simulink library "linkage_bushing_5DOF_lib"  (R2025a)
settings: Solver=VariableStepAuto  StartTime=0.0  StopTime=10.0  RelTol=1e-3
undefined symbols (not defined in the file): Bushing, Linear, Table, Visual, X, Y, Z
libraries: sm_lib x13, bushing_forces_lib x2
Description:
  | Component of Simscape Vehicle Templates Library
  | 
  | Copyright 2018-2025 The MathWorks, Inc.
settings Model: Creator=smiller  LastModifiedBy=smiller
settings OptimizationCC: ReuseModelBlockBuffer=off
settings ModelReferenceCC: EnableRefExpFcnMdlSchedulingChecks=on
settings RTWCC: GPUComputeCapability=3.5

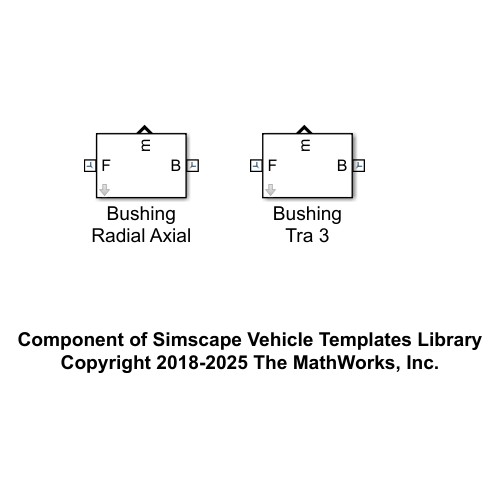
[thumbnail: Simulink's stored preview of the top-level diagram]
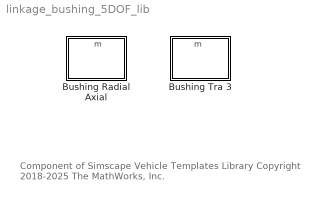
== system linkage_bushing_5DOF_lib ==
  note: Component of Simscape Vehicle Templates Library
      | Copyright 2018-2025 The MathWorks, Inc.
  Bushing Radial Axial : Subsystem  mask(Bushing with Radial and Axial Compliance){checkbox_setTargets=on, popup_force_law_spr_rad=Linear, k_radial=Bushing.RadialSpring.Linear.K.Value, x_radial=Bushing.RadialSpring.Table.x.Value, f_radial_spr=Bushing.RadialSpring.Table.f.Value, k1_radial_max=Bushing.RadialSpring.Maxwell.k1.Value, b1_radial_max=Bushing.RadialSpring.Maxwell.b1.Value, x_radial_max=Bushing.RadialSpring.Maxwell.x.Value, f_radial_max=Bushing.RadialSpring.Maxwell.f.Value, popup_force_law_dam_rad=Linear, d_radial=Bushing.RadialDamper.Linear.d.Value, v_radial=Bushing.RadialDamper.Table.v.Value, f_radial_dam=Bushing.RadialDamper.Table.f.Value, popup_force_law_spr_axi=Table, k_axial=Bushing.AxialSpring.Linear.K.Value, x_axial=Bushing.AxialSpring.Table.x.Value, f_axial_spr=Bushing.AxialSpring.Table.f.Value, popup_force_law_dam_axi=Table, d_axial=Bushing.AxialDamper.Linear.d.Value, v_axial=Bushing.AxialDamper.Linear.v.Value, f_axial_dam=Bushing.AxialDamper.Linear.f.Value, shell_or=Visual.hp.rad*1.05, shell_ir=Visual.hp.rad, shell_len=Visual.hp.rad*4, shell_clr=[0.5 0.5 0.5], shell_opc=1}
      mask prompts: checkbox_setTargets "Set position targets to 0"; popup_force_law_spr_rad "Spring Force Law"; k_radial "Spring Coefficient (N/mm)"; x_radial "Spring Deflection [min max] (mm)"; f_radial_spr "Spring Force [min max] (N)"; k1_radial_max "Maxwell k1"; b1_radial_max "Maxwell b1"; x_radial_max "Maxwell Displacement [min max] (mm)"; f_radial_max "Maxwell Force [min max] (N)"; popup_force_law_dam_rad "Damper Force Law"; d_radial "Damper Coefficient (N/(m/s))"; v_radial "Damper Velocity [min max] (m/s)"; f_radial_dam "Damper Force [min max] (N)"; popup_force_law_spr_axi "Spring Force Law"; k_axial "Spring Coefficient (N/mm)"; x_axial "Spring Displacement [min max] (mm)"; f_axial_spr "Spring Force [min max] (N)"; popup_force_law_dam_axi "Damper Force Law"; d_axial "Damper Coefficient (N/(m/s))"; v_axial "Damper Velocity [min max] (m/s)"; f_axial_dam "Damper Force [min max] (N)"; shell_or "Shell Outer Radius (m)"; shell_ir "Shell Inner Radius (m)"; shell_len "Shell Length (m)"; shell_clr "Shell Color [R G B]"; shell_opc "Shell Opacity [R G B]"
      mask help: Models bushing compliance with independent force laws for radial (x-y plane) and axial (z-axis) directions. Select force laws that model compliance as linear, nonlinear, or nonlinear with hysteresis. Only 5 degrees of freedom are permitted so that the connected part does not rotate about the axis connecting both ends.
      mask init:
      | if(checkbox_setTargets)
      |     set_param([gcb '/Bushing Joint'],...
      |         'PxPositionTargetSpecify','on',...
      |         'PyPositionTargetSpecify','on',...
      |         'PzPositionTargetSpecify','on'...
      |         );
      | else
      |     set_param([gcb '/Bushing Joint'],...
      |         'PxPositionTargetSpecify','off',...
      |         'PyPositionTargetSpecify','off',...
      |         'PzPositionTargetSpecify','off'...
      |         );
      | end
      settings: PortSchema="{\"entries\":[{\"content\":{\"sides\":[{\"content\":{\"connectorIds\":[\"LConn1\"]},\"type\":\"ConnectorPlacement.EquallySpacedRectSide\",\"uuid\":\"540bb151-3239-4a9d-82ba-b7afa97281a8\"},{\"content\":{\"connectorIds\":[\"RConn1\"],\"side\":\"RIGHT\"},\"type\":\"ConnectorPlacement.EquallySpacedRectSide\",\"uuid\":\"0af2999e-e304-4113-9c38-08ac5dd2068d\"},{\"content\":{\"connectorIds\":[\"Out1\"],\"side\":\"TOP\"},\"type\":\"ConnectorPlacement.EquallySpacedRectSide\",\"uuid\":\"c7e19545-6bd3-4656-b994-719fb436eca6\"}]},\"type\":\"ConnectorPlacement.EquallySpacedConnector\",\"uuid\":\"c532a1d4-44be-42d7-8101-c903e69d0a9b\"}],\"packageUris\":[\"http://schema.mathworks.com/mf0/Connector/R2020b\"],\"version\":\"1.0\"}"
      mask TypeOptions popup_force_law_spr_rad: Force Law/popup_force_law_spr_rad
      mask Callback popup_force_law_spr_rad:
      | maskObj = Simulink.Mask.get(gcb); % Get the mask object of the current block
      | krad_h  = maskObj.getParameter('k_radial'); % Get the parameter to hide
      | 
      | xrad_h  = maskObj.getParameter('x_radial'); % Get the parameter to hide
      | fSrad_h = maskObj.getParameter('f_radial_spr'); % Get the parameter to hide
      | k1rad_h  = maskObj.getParameter('k1_radial_max'); % Get the parameter to hide
      | b1rad_h  = maskObj.getParameter('b1_radial_max'); % Get the parameter to hide
      | xmrad_h  = maskObj.getParameter('x_radial_max'); % Get the parameter to hide
      | fmrad_h  = maskObj.getParameter('f_radial_max'); % Get the parameter to hide
      | 
      | % Check the value of ControlParam
      | frcLawSpr = get_param(gcb, 'popup_force_law_spr_rad');
      | 
      | krad_h.Visible  = 'off';
      | xrad_h.Visible  = 'off';
      | fSrad_h.Visible = 'off';
      | k1rad_h.Visible  = 'off';
      | b1rad_h.Visible  = 'off';
      | xmrad_h.Visible  = 'off';
      | fmrad_h.Visible  = 'off';
      | 
      | if strcmp(frcLawSpr, 'Linear')
      |     krad_h.Visible  = 'on';
      | elseif strcmp(frcLawSpr, 'Table')
      |     xrad_h.Visible  = 'on';
      |     fSrad_h.Visible = 'on';
      | elseif strcmp(frcLawSpr, 'Maxwell_SLS')
      |     k1rad_h.Visible  = 'on';
      |     b1rad_h.Visible = 'on';
      |     xmrad_h.Visible = 'on';
      |     fmrad_h.Visible = 'on';
      | end
      mask TypeOptions k_radial: Force Law/k_radial
      mask TypeOptions x_radial: Force Law/x_radial
      mask TypeOptions f_radial_spr: Force Law/f_radial_spr
      mask TypeOptions k1_radial_max: Force Law/k1_radial_max
      mask TypeOptions b1_radial_max: Force Law/b1_radial_max
      mask TypeOptions x_radial_max: Force Law/x_radial_max
      mask TypeOptions f_radial_max: Force Law/f_radial_max
      mask TypeOptions popup_force_law_dam_rad: Force Law/popup_force_law_dam_rad
      mask Callback popup_force_law_dam_rad:
      | maskObj = Simulink.Mask.get(gcb); % Get the mask object of the current block
      | drad_h  = maskObj.getParameter('d_radial'); % Get the parameter to hide
      | 
      | vrad_h  = maskObj.getParameter('v_radial'); % Get the parameter to hide
      | fDrad_h = maskObj.getParameter('f_radial_dam'); % Get the parameter to hide
      | 
      | % Check the value of ControlParam
      | frcLawDam = get_param(gcb, 'popup_force_law_dam_rad');
      | 
      | drad_h.Visible  = 'off';
      | vrad_h.Visible  = 'off';
      | fDrad_h.Visible = 'off';
      | 
      | if strcmp(frcLawDam, 'Linear')
      |     drad_h.Visible  = 'on';
      | elseif strcmp(frcLawDam, 'Table')
      |     vrad_h.Visible  = 'on';
      |     fDrad_h.Visible = 'on';
      | end
      mask TypeOptions d_radial: Force Law/d_radial
      mask TypeOptions v_radial: Force Law/v_radial
      mask TypeOptions f_radial_dam: Force Law/f_radial_dam
      mask TypeOptions popup_force_law_spr_axi: Force Law/popup_force_law_spr_axi
      mask Callback popup_force_law_spr_axi:
      | maskObj = Simulink.Mask.get(gcb); % Get the mask object of the current block
      | kaxi_h  = maskObj.getParameter('k_axial'); % Get the parameter to hide
      | 
      | xaxi_h  = maskObj.getParameter('x_axial'); % Get the parameter to hide
      | fSaxi_h  = maskObj.getParameter('f_axial_spr'); % Get the parameter to hide
      | 
      | % Check the value of ControlParam
      | controlParamValue = get_param(gcb, 'popup_force_law_spr_axi');
      | 
      | kaxi_h.Visible  = 'off';
      | xaxi_h.Visible  = 'off';
      | fSaxi_h.Visible  = 'off';
      | 
      | if strcmp(controlParamValue, 'Linear')
      |     kaxi_h.Visible  = 'on';
      | else
      |     xaxi_h.Visible  = 'on';
      |     fSaxi_h.Visible  = 'on';
      | end
      mask TypeOptions k_axial: Force Law/k_axial
      mask TypeOptions x_axial: Force Law/x_axial
      mask TypeOptions f_axial_spr: Force Law/f_axial_spr
      mask TypeOptions popup_force_law_dam_axi: Force Law/popup_force_law_dam_axi
      mask Callback popup_force_law_dam_axi:
      | maskObj = Simulink.Mask.get(gcb); % Get the mask object of the current block
      | daxi_h  = maskObj.getParameter('d_axial'); % Get the parameter to hide
      | 
      | vaxi_h  = maskObj.getParameter('v_axial'); % Get the parameter to hide
      | fDaxi_h  = maskObj.getParameter('f_axial_dam'); % Get the parameter to hide
      | 
      | % Check the value of ControlParam
      | controlParamValue = get_param(gcb, 'popup_force_law_dam_axi');
      | 
      | daxi_h.Visible  = 'off';
      | vaxi_h.Visible  = 'off';
      | fDaxi_h.Visible  = 'off';
      | 
      | if strcmp(controlParamValue, 'Linear')
      |     daxi_h.Visible  = 'on';
      | else
      |     vaxi_h.Visible  = 'on';
      |     fDaxi_h.Visible  = 'on';
      | end
      mask TypeOptions d_axial: Force Law/d_axial
      mask TypeOptions v_axial: Force Law/v_axial
      mask TypeOptions f_axial_dam: Force Law/f_axial_dam
      mask DialogControl cont_radial Prompt: Radial
      mask DialogControl cont_axial Prompt: Axial
      mask DialogControl cont_vis Prompt: Visualization
  Bushing Tra 3 : Subsystem  mask(Bushing with Independent Axial Compliance on 3 Axes (5 DOF)){checkbox_setTargets=on, popup_force_law_spr_axiX=Linear, k_axialX=Bushing.SpringX.Linear.K.Value, x_axialX=Bushing.SpringX.Table.x.Value, f_axialX_spr=Bushing.SpringX.Table.f.Value, popup_force_law_dam_axiX=Linear, d_axialX=Bushing.DamperX.Linear.d.Value, v_axialX=Bushing.DamperX.Table.v.Value, f_axialX_dam=Bushing.DamperX.Table.f.Value, popup_force_law_spr_axiY=Linear, k_axialY=Bushing.SpringY.Linear.K.Value, x_axialY=Bushing.SpringY.Table.x.Value, f_axialY_spr=Bushing.SpringY.Table.f.Value, popup_force_law_dam_axiY=Linear, d_axialY=Bushing.DamperY.Linear.d.Value, v_axialY=Bushing.DamperY.Table.v.Value, f_axialY_dam=Bushing.DamperY.Table.f.Value, popup_force_law_spr_axiZ=Table, k_axialZ=Bushing.SpringZ.Linear.K.Value, x_axialZ=Bushing.SpringZ.Table.x.Value, f_axialZ_spr=Bushing.SpringZ.Table.f.Value, popup_force_law_dam_axiZ=Table, d_axialZ=Bushing.DamperZ.Linear.d.Value, v_axialZ=Bushing.DamperZ.Table.v.Value, f_axialZ_dam=Bushing.DamperZ.Table.f.Value, shell_or=Visual.hp.rad*2, shell_ir=Visual.hp.rad, shell_len=Visual.hp.rad*2, shell_clr=Visual.Bushing.clr, shell_opc=Visual.part.opc}
      mask prompts: checkbox_setTargets "Set position targets to 0"; popup_force_law_spr_axiX "Spring Force Law"; k_axialX "Spring Coefficient (N/mm)"; x_axialX "Spring Displacement [min max] (mm)"; f_axialX_spr "Spring Force [min max] (N)"; popup_force_law_dam_axiX "Damper Force Law"; d_axialX "Damper Coefficient (N/(m/s))"; v_axialX "Damper Velocity [min max] (m/s)"; f_axialX_dam "Damper Force [min max] (N)"; popup_force_law_spr_axiY "Spring Force Law"; k_axialY "Spring Coefficient (N/mm)"; x_axialY "Spring Displacement [min max] (mm)"; f_axialY_spr "Spring Force [min max] (N)"; popup_force_law_dam_axiY "Damper Force Law"; d_axialY "Damper Coefficient (N/(m/s))"; v_axialY "Damper Velocity [min max] (m/s)"; f_axialY_dam "Damper Force [min max] (N)"; popup_force_law_spr_axiZ "Spring Force Law"; k_axialZ "Spring Coefficient (N/mm)"; x_axialZ "Spring Displacement [min max] (mm)"; f_axialZ_spr "Spring Force [min max] (N)"; popup_force_law_dam_axiZ "Damper Force Law"; d_axialZ "Damper Coefficient (N/(m/s))"; v_axialZ "Damper Velocity [min max] (m/s)"; f_axialZ_dam "Damper Force [min max] (N)"; shell_or "Shell Outer Radius (m)"; shell_ir "Shell Inner Radius (m)"; shell_len "Shell Length (m)"; shell_clr "Shell Color [R G B]"; shell_opc "Shell Opacity [R G B]"
      mask help: Models bushing compliance with independent force laws for x, y, and z directions. Select force laws that model compliance as linear, nonlinear, or nonlinear with hysteresis. Only 5 degrees of freedom are permitted so that the connected part does not rotate about the axis connecting both ends.
      mask init: same as linkage_bushing_5DOF_lib/Bushing Radial Axial
      settings: PortSchema="{\"entries\":[{\"content\":{\"sides\":[{\"content\":{\"connectorIds\":[\"LConn1\"]},\"type\":\"ConnectorPlacement.EquallySpacedRectSide\",\"uuid\":\"540bb151-3239-4a9d-82ba-b7afa97281a8\"},{\"content\":{\"connectorIds\":[\"RConn1\"],\"side\":\"RIGHT\"},\"type\":\"ConnectorPlacement.EquallySpacedRectSide\",\"uuid\":\"0af2999e-e304-4113-9c38-08ac5dd2068d\"},{\"content\":{\"connectorIds\":[\"Out1\"],\"side\":\"TOP\"},\"type\":\"ConnectorPlacement.EquallySpacedRectSide\",\"uuid\":\"c7e19545-6bd3-4656-b994-719fb436eca6\"}]},\"type\":\"ConnectorPlacement.EquallySpacedConnector\",\"uuid\":\"c532a1d4-44be-42d7-8101-c903e69d0a9b\"}],\"packageUris\":[\"http://schema.mathworks.com/mf0/Connector/R2020b\"],\"version\":\"1.0\"}"
      mask TypeOptions popup_force_law_spr_axiX: Force Law/popup_force_law_spr_axiX
      mask Callback popup_force_law_spr_axiX:
      | maskObj = Simulink.Mask.get(gcb); % Get the mask object of the current block
      | kaxiX_h  = maskObj.getParameter('k_axialX'); % Get the parameter to hide
      | 
      | xaxiX_h  = maskObj.getParameter('x_axialX'); % Get the parameter to hide
      | fSaxiX_h  = maskObj.getParameter('f_axialX_spr'); % Get the parameter to hide
      | 
      | % Check the value of ControlParam
      | controlParamValue = get_param(gcb, 'popup_force_law_spr_axiX');
      | 
      | kaxiX_h.Visible  = 'off';
      | xaxiX_h.Visible  = 'off';
      | fSaxiX_h.Visible  = 'off';
      | 
      | if strcmp(controlParamValue, 'Linear')
      |     kaxiX_h.Visible  = 'on';
      | else
      |     xaxiX_h.Visible  = 'on';
      |     fSaxiX_h.Visible  = 'on';
      | end
      mask TypeOptions k_axialX: Force Law/k_axialX
      mask TypeOptions x_axialX: Force Law/x_axialX
      mask TypeOptions f_axialX_spr: Force Law/f_axialX_spr
      mask TypeOptions popup_force_law_dam_axiX: Force Law/popup_force_law_dam_axiX
      mask Callback popup_force_law_dam_axiX:
      | maskObj = Simulink.Mask.get(gcb); % Get the mask object of the current block
      | daxiX_h  = maskObj.getParameter('d_axialX'); % Get the parameter to hide
      | 
      | vaxiX_h  = maskObj.getParameter('v_axialX'); % Get the parameter to hide
      | fDaxiX_h  = maskObj.getParameter('f_axialX_dam'); % Get the parameter to hide
      | 
      | % Check the value of ControlParam
      | controlParamValue = get_param(gcb, 'popup_force_law_dam_axiX');
      | 
      | daxiX_h.Visible  = 'off';
      | vaxiX_h.Visible  = 'off';
      | fDaxiX_h.Visible  = 'off';
      | 
      | if strcmp(controlParamValue, 'Linear')
      |     daxiX_h.Visible  = 'on';
      | else
      |     vaxiX_h.Visible  = 'on';
      |     fDaxiX_h.Visible  = 'on';
      | end
      mask TypeOptions d_axialX: Force Law/d_axialX
      mask TypeOptions v_axialX: Force Law/v_axialX
      mask TypeOptions f_axialX_dam: Force Law/f_axialX_dam
      mask TypeOptions popup_force_law_spr_axiY: Force Law/popup_force_law_spr_axiY
      mask Callback popup_force_law_spr_axiY:
      | maskObj = Simulink.Mask.get(gcb); % Get the mask object of the current block
      | kaxiY_h  = maskObj.getParameter('k_axialY'); % Get the parameter to hide
      | 
      | xaxiY_h  = maskObj.getParameter('x_axialY'); % Get the parameter to hide
      | fSaxiY_h  = maskObj.getParameter('f_axialY_spr'); % Get the parameter to hide
      | 
      | % Check the value of ControlParam
      | controlParamValue = get_param(gcb, 'popup_force_law_spr_axiY');
      | 
      | kaxiY_h.Visible  = 'off';
      | xaxiY_h.Visible  = 'off';
      | fSaxiY_h.Visible  = 'off';
      | 
      | if strcmp(controlParamValue, 'Linear')
      |     kaxiY_h.Visible  = 'on';
      | else
      |     xaxiY_h.Visible  = 'on';
      |     fSaxiY_h.Visible  = 'on';
      | end
      mask TypeOptions k_axialY: Force Law/k_axialY
      mask TypeOptions x_axialY: Force Law/x_axialY
      mask TypeOptions f_axialY_spr: Force Law/f_axialY_spr
      mask TypeOptions popup_force_law_dam_axiY: Force Law/popup_force_law_dam_axiY
      mask Callback popup_force_law_dam_axiY:
      | maskObj = Simulink.Mask.get(gcb); % Get the mask object of the current block
      | daxiY_h  = maskObj.getParameter('d_axialY'); % Get the parameter to hide
      | 
      | vaxiY_h  = maskObj.getParameter('v_axialY'); % Get the parameter to hide
      | fDaxiY_h  = maskObj.getParameter('f_axialY_dam'); % Get the parameter to hide
      | 
      | % Check the value of ControlParam
      | controlParamValue = get_param(gcb, 'popup_force_law_dam_axiY');
      | 
      | daxiY_h.Visible  = 'off';
      | vaxiY_h.Visible  = 'off';
      | fDaxiY_h.Visible  = 'off';
      | 
      | if strcmp(controlParamValue, 'Linear')
      |     daxiY_h.Visible  = 'on';
      | else
      |     vaxiY_h.Visible  = 'on';
      |     fDaxiY_h.Visible  = 'on';
      | end
      mask TypeOptions d_axialY: Force Law/d_axialY
      mask TypeOptions v_axialY: Force Law/v_axialY
      mask TypeOptions f_axialY_dam: Force Law/f_axialY_dam
      mask TypeOptions popup_force_law_spr_axiZ: Force Law/popup_force_law_spr_axiZ
      mask Callback popup_force_law_spr_axiZ:
      | maskObj = Simulink.Mask.get(gcb); % Get the mask object of the current block
      | kaxiZ_h  = maskObj.getParameter('k_axialZ'); % Get the parameter to hide
      | 
      | xaxiZ_h  = maskObj.getParameter('x_axialZ'); % Get the parameter to hide
      | fSaxiZ_h  = maskObj.getParameter('f_axialZ_spr'); % Get the parameter to hide
      | 
      | % Check the value of ControlParam
      | controlParamValue = get_param(gcb, 'popup_force_law_spr_axiZ');
      | 
      | kaxiZ_h.Visible  = 'off';
      | xaxiZ_h.Visible  = 'off';
      | fSaxiZ_h.Visible  = 'off';
      | 
      | if strcmp(controlParamValue, 'Linear')
      |     kaxiZ_h.Visible  = 'on';
      | else
      |     xaxiZ_h.Visible  = 'on';
      |     fSaxiZ_h.Visible  = 'on';
      | end
      mask TypeOptions k_axialZ: Force Law/k_axialZ
      mask TypeOptions x_axialZ: Force Law/x_axialZ
      mask TypeOptions f_axialZ_spr: Force Law/f_axialZ_spr
      mask TypeOptions popup_force_law_dam_axiZ: Force Law/popup_force_law_dam_axiZ
      mask Callback popup_force_law_dam_axiZ:
      | maskObj = Simulink.Mask.get(gcb); % Get the mask object of the current block
      | daxiZ_h  = maskObj.getParameter('d_axialZ'); % Get the parameter to hide
      | 
      | vaxiZ_h  = maskObj.getParameter('v_axialZ'); % Get the parameter to hide
      | fDaxiZ_h  = maskObj.getParameter('f_axialZ_dam'); % Get the parameter to hide
      | 
      | % Check the value of ControlParam
      | controlParamValue = get_param(gcb, 'popup_force_law_dam_axiZ');
      | 
      | daxiZ_h.Visible  = 'off';
      | vaxiZ_h.Visible  = 'off';
      | fDaxiZ_h.Visible  = 'off';
      | 
      | if strcmp(controlParamValue, 'Linear')
      |     daxiZ_h.Visible  = 'on';
      | else
      |     vaxiZ_h.Visible  = 'on';
      |     fDaxiZ_h.Visible  = 'on';
      | end
      mask TypeOptions d_axialZ: Force Law/d_axialZ
      mask TypeOptions v_axialZ: Force Law/v_axialZ
      mask TypeOptions f_axialZ_dam: Force Law/f_axialZ_dam
      mask DialogControl cont_axialX Prompt: Axial (local x)
      mask DialogControl cont_axialY Prompt: Axial (local y)
      mask DialogControl cont_axialZ Prompt: Axial (local z)
      mask DialogControl cont_vis Prompt: Visualization

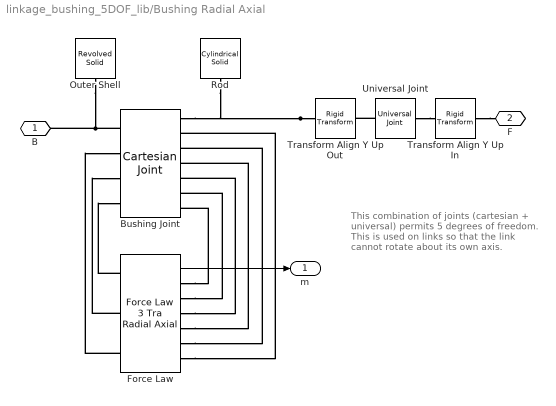
== system linkage_bushing_5DOF_lib/Bushing Radial Axial ==
  note: This combination of joints (cartesian + universal) permits 5 degrees of freedom. This is used on links so that the link cannot rotate about its own axis.
  Bushing Joint : sm_lib/Joints/Cartesian Joint  JointMode=Normal  CompositeWrenchDir=FollowerOnBase  CompositeWrenchFrame=BaseFrame  SenseConstraintForce=off  SenseConstraintTorque=off  SenseTotalForce=off  SenseTotalTorque=off  PxPositionTargetSpecify=on  PxPositionTargetPriority=High  PxPositionTargetValue=0  PxPositionTargetValueUnits=m  PxVelocityTargetSpecify=off  PxVelocityTargetPriority=High  PxVelocityTargetValue=0  PxVelocityTargetValueUnits=m/s  PxEquilibriumPosition=0  PxEquilibriumPositionUnits=m  PxSpringStiffness=0  PxSpringStiffnessUnits=N/m  PxDampingCoefficient=0  PxDampingCoefficientUnits=N/(m/s)  PxLowerLimitSpecify=off  PxLowerLimitBound=-1  PxLowerLimitBoundUnits=m  PxLowerLimitStiffness=1e6  PxLowerLimitStiffnessUnits=N/m  PxLowerLimitDamping=1e3  PxLowerLimitDampingUnits=N/(m/s)  PxLowerLimitTransitionRegionWidth=1e-4  PxLowerLimitTransitionRegionWidthUnits=m  PxUpperLimitSpecify=off  PxUpperLimitBound=1  PxUpperLimitBoundUnits=m  PxUpperLimitStiffness=1e6  PxUpperLimitStiffnessUnits=N/m  PxUpperLimitDamping=1e3  PxUpperLimitDampingUnits=N/(m/s)  PxUpperLimitTransitionRegionWidth=1e-4  PxUpperLimitTransitionRegionWidthUnits=m  PxTorqueActuationMode=InputTorque  PxMotionActuationMode=ComputedMotion  PxSensePosition=on  PxSenseVelocity=on  PxSenseAcceleration=off  PxSenseTorqueForce=off  PxSenseLowerLimitTorqueForce=off  PxSenseUpperLimitTorqueForce=off  PyPositionTargetSpecify=on  PyPositionTargetPriority=High  PyPositionTargetValue=0  PyPositionTargetValueUnits=m  PyVelocityTargetSpecify=off  PyVelocityTargetPriority=High  PyVelocityTargetValue=0  PyVelocityTargetValueUnits=m/s  PyEquilibriumPosition=0  PyEquilibriumPositionUnits=m  PySpringStiffness=0  PySpringStiffnessUnits=N/m  PyDampingCoefficient=0  PyDampingCoefficientUnits=N/(m/s)  PyLowerLimitSpecify=off  PyLowerLimitBound=-1  PyLowerLimitBoundUnits=m  PyLowerLimitStiffness=1e6  PyLowerLimitStiffnessUnits=N/m  PyLowerLimitDamping=1e3  PyLowerLimitDampingUnits=N/(m/s)  PyLowerLimitTransitionRegionWidth=1e-4  PyLowerLimitTransitionRegionWidthUnits=m  PyUpperLimitSpecify=off  PyUpperLimitBound=1  PyUpperLimitBoundUnits=m  PyUpperLimitStiffness=1e6  PyUpperLimitStiffnessUnits=N/m  PyUpperLimitDamping=1e3  PyUpperLimitDampingUnits=N/(m/s)  PyUpperLimitTransitionRegionWidth=1e-4  PyUpperLimitTransitionRegionWidthUnits=m  PyTorqueActuationMode=InputTorque  PyMotionActuationMode=ComputedMotion  PySensePosition=on  PySenseVelocity=on  PySenseAcceleration=off  PySenseTorqueForce=off  PySenseLowerLimitTorqueForce=off  PySenseUpperLimitTorqueForce=off  PzPositionTargetSpecify=on  PzPositionTargetPriority=High  PzPositionTargetValue=0  PzPositionTargetValueUnits=m  PzVelocityTargetSpecify=off  PzVelocityTargetPriority=High  PzVelocityTargetValue=0  PzVelocityTargetValueUnits=m/s  PzEquilibriumPosition=0  PzEquilibriumPositionUnits=m  PzSpringStiffness=0  PzSpringStiffnessUnits=N/m  PzDampingCoefficient=0  PzDampingCoefficientUnits=N/(m/s)  PzLowerLimitSpecify=off  PzLowerLimitBound=-1  PzLowerLimitBoundUnits=m  PzLowerLimitStiffness=1e6  PzLowerLimitStiffnessUnits=N/m  PzLowerLimitDamping=1e3  PzLowerLimitDampingUnits=N/(m/s)  PzLowerLimitTransitionRegionWidth=1e-4  PzLowerLimitTransitionRegionWidthUnits=m  PzUpperLimitSpecify=off  PzUpperLimitBound=1  PzUpperLimitBoundUnits=m  PzUpperLimitStiffness=1e6  PzUpperLimitStiffnessUnits=N/m  PzUpperLimitDamping=1e3  PzUpperLimitDampingUnits=N/(m/s)  PzUpperLimitTransitionRegionWidth=1e-4  PzUpperLimitTransitionRegionWidthUnits=m  PzTorqueActuationMode=InputTorque  PzMotionActuationMode=ComputedMotion  PzSensePosition=on  PzSenseVelocity=on  PzSenseAcceleration=off  PzSenseTorqueForce=off  PzSenseLowerLimitTorqueForce=off  PzSenseUpperLimitTorqueForce=off
  Force Law : bushing_forces_lib/Force Law 3 Tra Radial Axial  popup_force_law_spr_rad=Linear  k_radial=k_radial  x_radial=x_radial  f_radial_spr=f_radial_spr  k1_radial_max=k1_radial_max  b1_radial_max=b1_radial_max  x_radial_max=x_radial_max  f_radial_max=f_radial_max  popup_force_law_dam_rad=Linear  d_radial=d_radial  v_radial=v_radial  f_radial_dam=f_radial_dam  popup_force_law_spr_axi=Table  k_axial=k_axial  x_axial=x_axial  f_axial_spr=f_axial_spr  popup_force_law_dam_axi=Table  d_axial=d_axial  v_axial=v_axial  f_axial_dam=f_axial_dam
  Outer Shell : sm_lib/Body Elements/Revolved Solid  RevolutionCrossSection=[shell_ir 0.5; shell_ir -0.5; shell_or -0.5; shell_or 0.5].*[1 shell_len]  RevolutionCrossSectionUnits=m  RevolutionExtent=Full  RevolutionAngle=180  RevolutionAngleUnits=deg  ExportConvexHullGeometry=off  InertiaType=CalculateFromGeometry  BasedOnType=Density  Density=1  DensityUnits=kg/m^3  Mass=1  MassUnits=kg  CenterOfMass=[0 0 0]  CenterOfMassUnits=m  MomentsOfInertia=[1 1 1]  MomentsOfInertiaUnits=kg*m^2  ProductsOfInertia=[0 0 0]  ProductsOfInertiaUnits=kg*m^2  GraphicType=FromGeometry  MarkerShape=Sphere  MarkerSize=10  GraphicVisPropType=SimpleVisualProperties  GraphicDiffuseColor=shell_clr  GraphicOpacity=shell_opc  GraphicSpecularColor=[0.5 0.5 0.5 1.0]  GraphicAmbientColor=[0.15 0.15 0.15 1.0]  GraphicEmissiveColor=[0.0 0.0 0.0 1.0]  GraphicShininess=75  DoExposeReferenceFrame=on  SerializedFrames=<Frames/>
  Rod : sm_lib/Body Elements/Cylindrical Solid  CylinderRadius=shell_ir/2  CylinderRadiusUnits=m  CylinderLength=shell_len  CylinderLengthUnits=m  ExportEntireGeometry=off  InertiaType=CalculateFromGeometry  BasedOnType=Density  Density=1  DensityUnits=kg/m^3  Mass=1  MassUnits=kg  CenterOfMass=[0 0 0]  CenterOfMassUnits=m  MomentsOfInertia=[1 1 1]  MomentsOfInertiaUnits=kg*m^2  ProductsOfInertia=[0 0 0]  ProductsOfInertiaUnits=kg*m^2  GraphicType=FromGeometry  MarkerShape=Sphere  MarkerSize=10  GraphicVisPropType=SimpleVisualProperties  GraphicDiffuseColor=shell_clr  GraphicOpacity=shell_opc  GraphicSpecularColor=[0.5 0.5 0.5 1.0]  GraphicAmbientColor=[0.15 0.15 0.15 1.0]  GraphicEmissiveColor=[0.0 0.0 0.0 1.0]  GraphicShininess=75  DoExposeReferenceFrame=on  SerializedFrames=<Frames/>
  Transform Align Y Up In : sm_lib/Frames and Transforms/Rigid Transform  RotationMethod=StandardAxis  FollAlignAxisA=+X  BaseAlignAxisA=+Y  FollAlignAxisB=+Y  BaseAlignAxisB=+Z  RotationStandardAxis=+X  RotationAngle=90  RotationAngleUnits=deg  RotationArbitraryAxis=[0 0 1]  RotationSequenceAxes=FollowerAxes  RotationSequence=XYX  RotationSequenceAngles=[0 0 0]  RotationSequenceAnglesUnits=deg  RotationMatrix=[1 0 0; 0 1 0; 0 0 1]  Quaternion=[1 0 0 0]  TranslationMethod=None  TranslationCartesianOffset=[0 0 0]  TranslationCartesianOffsetUnits=m  TranslationStandardAxis=+Z  TranslationStandardOffset=0  TranslationStandardOffsetUnits=m  TranslationROffset=0  TranslationROffsetUnits=m  TranslationThetaOffset=0  TranslationThetaOffsetUnits=deg  TranslationZOffset=0  TranslationZOffsetUnits=m
  Transform Align Y Up Out : sm_lib/Frames and Transforms/Rigid Transform  RotationMethod=StandardAxis  FollAlignAxisA=+X  BaseAlignAxisA=+Y  FollAlignAxisB=+Y  BaseAlignAxisB=+Z  RotationStandardAxis=+X  RotationAngle=90  RotationAngleUnits=deg  RotationArbitraryAxis=[0 0 1]  RotationSequenceAxes=FollowerAxes  RotationSequence=XYX  RotationSequenceAngles=[0 0 0]  RotationSequenceAnglesUnits=deg  RotationMatrix=[1 0 0; 0 1 0; 0 0 1]  Quaternion=[1 0 0 0]  TranslationMethod=None  TranslationCartesianOffset=[0 0 0]  TranslationCartesianOffsetUnits=m  TranslationStandardAxis=+Z  TranslationStandardOffset=0  TranslationStandardOffsetUnits=m  TranslationROffset=0  TranslationROffsetUnits=m  TranslationThetaOffset=0  TranslationThetaOffsetUnits=deg  TranslationZOffset=0  TranslationZOffsetUnits=m
  Universal Joint : sm_lib/Joints/Universal Joint  JointMode=Normal  CompositeWrenchDir=FollowerOnBase  CompositeWrenchFrame=BaseFrame  SenseConstraintForce=off  SenseConstraintTorque=off  SenseTotalForce=off  SenseTotalTorque=off  RxPositionTargetSpecify=off  RxPositionTargetPriority=High  RxPositionTargetValue=0  RxPositionTargetValueUnits=deg  RxVelocityTargetSpecify=off  RxVelocityTargetPriority=High  RxVelocityTargetValue=0  RxVelocityTargetValueUnits=deg/s  RxEquilibriumPosition=0  RxEquilibriumPositionUnits=deg  RxSpringStiffness=0  RxSpringStiffnessUnits=N*m/deg  RxDampingCoefficient=0  RxDampingCoefficientUnits=N*m/(deg/s)  RxLowerLimitSpecify=off  RxLowerLimitBound=-90  RxLowerLimitBoundUnits=deg  RxLowerLimitStiffness=1e4  RxLowerLimitStiffnessUnits=N*m/deg  RxLowerLimitDamping=10  RxLowerLimitDampingUnits=N*m/(deg/s)  RxLowerLimitTransitionRegionWidth=0.1  RxLowerLimitTransitionRegionWidthUnits=deg  RxUpperLimitSpecify=off  RxUpperLimitBound=90  RxUpperLimitBoundUnits=deg  RxUpperLimitStiffness=1e4  RxUpperLimitStiffnessUnits=N*m/deg  RxUpperLimitDamping=10  RxUpperLimitDampingUnits=N*m/(deg/s)  RxUpperLimitTransitionRegionWidth=0.1  RxUpperLimitTransitionRegionWidthUnits=deg  RxTorqueActuationMode=NoTorque  RxMotionActuationMode=ComputedMotion  RxSensePosition=off  RxSenseVelocity=off  RxSenseAcceleration=off  RxSenseTorqueForce=off  RxSenseLowerLimitTorqueForce=off  RxSenseUpperLimitTorqueForce=off  RyPositionTargetSpecify=off  RyPositionTargetPriority=High  RyPositionTargetValue=0  RyPositionTargetValueUnits=deg  RyVelocityTargetSpecify=off  RyVelocityTargetPriority=High  RyVelocityTargetValue=0  RyVelocityTargetValueUnits=deg/s  RyEquilibriumPosition=0  RyEquilibriumPositionUnits=deg  RySpringStiffness=0  RySpringStiffnessUnits=N*m/deg  RyDampingCoefficient=0  RyDampingCoefficientUnits=N*m/(deg/s)  RyLowerLimitSpecify=off  RyLowerLimitBound=-90  RyLowerLimitBoundUnits=deg  RyLowerLimitStiffness=1e4  RyLowerLimitStiffnessUnits=N*m/deg  RyLowerLimitDamping=10  RyLowerLimitDampingUnits=N*m/(deg/s)  RyLowerLimitTransitionRegionWidth=0.1  RyLowerLimitTransitionRegionWidthUnits=deg  RyUpperLimitSpecify=off  RyUpperLimitBound=90  RyUpperLimitBoundUnits=deg  RyUpperLimitStiffness=1e4  RyUpperLimitStiffnessUnits=N*m/deg  RyUpperLimitDamping=10  RyUpperLimitDampingUnits=N*m/(deg/s)  RyUpperLimitTransitionRegionWidth=0.1  RyUpperLimitTransitionRegionWidthUnits=deg  RyTorqueActuationMode=NoTorque  RyMotionActuationMode=ComputedMotion  RySensePosition=off  RySenseVelocity=off  RySenseAcceleration=off  RySenseTorqueForce=off  RySenseLowerLimitTorqueForce=off  RySenseUpperLimitTorqueForce=off
  B : PMIOPort  Side=Left
  F : PMIOPort  Port=2  Side=Right
  m : Outport
  wires:
  Force Law/1 -> m/1
  connections:
  Force Law/LConn2 -- Bushing Joint/LConn3
  Force Law/RConn5 -- Bushing Joint/RConn3
  Force Law/LConn3 -- Bushing Joint/LConn2
  Force Law/LConn1 -- Bushing Joint/LConn4
  Force Law/RConn1 -- Bushing Joint/RConn7
  Force Law/RConn3 -- Bushing Joint/RConn5
  Force Law/RConn2 -- Bushing Joint/RConn6
  Force Law/RConn4 -- Bushing Joint/RConn4
  Force Law/RConn6 -- Bushing Joint/RConn2
  Transform Align Y Up Out/LConn1 -- Bushing Joint/RConn1 -- Rod/RConn1
  Universal Joint/LConn1 -- Transform Align Y Up Out/RConn1
  Universal Joint/RConn1 -- Transform Align Y Up In/RConn1
  Outer Shell/RConn1 -- B/RConn1 -- Bushing Joint/LConn1
  Transform Align Y Up In/LConn1 -- F/RConn1

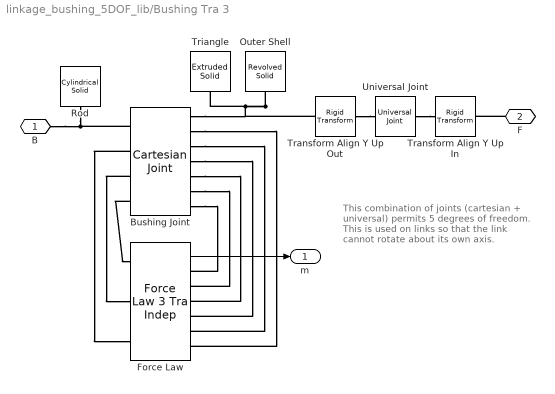
== system linkage_bushing_5DOF_lib/Bushing Tra 3 ==
  note: This combination of joints (cartesian + universal) permits 5 degrees of freedom. This is used on links so that the link cannot rotate about its own axis.
  Bushing Joint : sm_lib/Joints/Cartesian Joint  JointMode=Normal  CompositeWrenchDir=FollowerOnBase  CompositeWrenchFrame=BaseFrame  SenseConstraintForce=off  SenseConstraintTorque=off  SenseTotalForce=off  SenseTotalTorque=off  PxPositionTargetSpecify=on  PxPositionTargetPriority=High  PxPositionTargetValue=0  PxPositionTargetValueUnits=m  PxVelocityTargetSpecify=off  PxVelocityTargetPriority=High  PxVelocityTargetValue=0  PxVelocityTargetValueUnits=m/s  PxEquilibriumPosition=0  PxEquilibriumPositionUnits=m  PxSpringStiffness=0  PxSpringStiffnessUnits=N/m  PxDampingCoefficient=0  PxDampingCoefficientUnits=N/(m/s)  PxLowerLimitSpecify=off  PxLowerLimitBound=-1  PxLowerLimitBoundUnits=m  PxLowerLimitStiffness=1e6  PxLowerLimitStiffnessUnits=N/m  PxLowerLimitDamping=1e3  PxLowerLimitDampingUnits=N/(m/s)  PxLowerLimitTransitionRegionWidth=1e-4  PxLowerLimitTransitionRegionWidthUnits=m  PxUpperLimitSpecify=off  PxUpperLimitBound=1  PxUpperLimitBoundUnits=m  PxUpperLimitStiffness=1e6  PxUpperLimitStiffnessUnits=N/m  PxUpperLimitDamping=1e3  PxUpperLimitDampingUnits=N/(m/s)  PxUpperLimitTransitionRegionWidth=1e-4  PxUpperLimitTransitionRegionWidthUnits=m  PxTorqueActuationMode=InputTorque  PxMotionActuationMode=ComputedMotion  PxSensePosition=on  PxSenseVelocity=on  PxSenseAcceleration=off  PxSenseTorqueForce=off  PxSenseLowerLimitTorqueForce=off  PxSenseUpperLimitTorqueForce=off  PyPositionTargetSpecify=on  PyPositionTargetPriority=High  PyPositionTargetValue=0  PyPositionTargetValueUnits=m  PyVelocityTargetSpecify=off  PyVelocityTargetPriority=High  PyVelocityTargetValue=0  PyVelocityTargetValueUnits=m/s  PyEquilibriumPosition=0  PyEquilibriumPositionUnits=m  PySpringStiffness=0  PySpringStiffnessUnits=N/m  PyDampingCoefficient=0  PyDampingCoefficientUnits=N/(m/s)  PyLowerLimitSpecify=off  PyLowerLimitBound=-1  PyLowerLimitBoundUnits=m  PyLowerLimitStiffness=1e6  PyLowerLimitStiffnessUnits=N/m  PyLowerLimitDamping=1e3  PyLowerLimitDampingUnits=N/(m/s)  PyLowerLimitTransitionRegionWidth=1e-4  PyLowerLimitTransitionRegionWidthUnits=m  PyUpperLimitSpecify=off  PyUpperLimitBound=1  PyUpperLimitBoundUnits=m  PyUpperLimitStiffness=1e6  PyUpperLimitStiffnessUnits=N/m  PyUpperLimitDamping=1e3  PyUpperLimitDampingUnits=N/(m/s)  PyUpperLimitTransitionRegionWidth=1e-4  PyUpperLimitTransitionRegionWidthUnits=m  PyTorqueActuationMode=InputTorque  PyMotionActuationMode=ComputedMotion  PySensePosition=on  PySenseVelocity=on  PySenseAcceleration=off  PySenseTorqueForce=off  PySenseLowerLimitTorqueForce=off  PySenseUpperLimitTorqueForce=off  PzPositionTargetSpecify=on  PzPositionTargetPriority=High  PzPositionTargetValue=0  PzPositionTargetValueUnits=m  PzVelocityTargetSpecify=off  PzVelocityTargetPriority=High  PzVelocityTargetValue=0  PzVelocityTargetValueUnits=m/s  PzEquilibriumPosition=0  PzEquilibriumPositionUnits=m  PzSpringStiffness=0  PzSpringStiffnessUnits=N/m  PzDampingCoefficient=0  PzDampingCoefficientUnits=N/(m/s)  PzLowerLimitSpecify=off  PzLowerLimitBound=-1  PzLowerLimitBoundUnits=m  PzLowerLimitStiffness=1e6  PzLowerLimitStiffnessUnits=N/m  PzLowerLimitDamping=1e3  PzLowerLimitDampingUnits=N/(m/s)  PzLowerLimitTransitionRegionWidth=1e-4  PzLowerLimitTransitionRegionWidthUnits=m  PzUpperLimitSpecify=off  PzUpperLimitBound=1  PzUpperLimitBoundUnits=m  PzUpperLimitStiffness=1e6  PzUpperLimitStiffnessUnits=N/m  PzUpperLimitDamping=1e3  PzUpperLimitDampingUnits=N/(m/s)  PzUpperLimitTransitionRegionWidth=1e-4  PzUpperLimitTransitionRegionWidthUnits=m  PzTorqueActuationMode=InputTorque  PzMotionActuationMode=ComputedMotion  PzSensePosition=on  PzSenseVelocity=on  PzSenseAcceleration=off  PzSenseTorqueForce=off  PzSenseLowerLimitTorqueForce=off  PzSenseUpperLimitTorqueForce=off
  Force Law : bushing_forces_lib/Force Law 3 Tra Indep  popup_force_law_spr_axiX=Linear  k_axialX=k_axialX  x_axialX=x_axialX  f_axialX_spr=f_axialX_spr  popup_force_law_dam_axiX=Linear  d_axialX=d_axialX  v_axialX=v_axialX  f_axialX_dam=f_axialX_dam  popup_force_law_spr_axiY=Linear  k_axialY=k_axialY  x_axialY=x_axialY  f_axialY_spr=f_axialY_spr  popup_force_law_dam_axiY=Linear  d_axialY=d_axialY  v_axialY=v_axialY  f_axialY_dam=f_axialY_dam  popup_force_law_spr_axiZ=Table  k_axialZ=k_axialZ  x_axialZ=x_axialZ  f_axialZ_spr=f_axialZ_spr  popup_force_law_dam_axiZ=Table  d_axialZ=d_axialZ  f_axialZ_dam=f_axialZ_dam  v_axialZ=v_axialZ
  Outer Shell : sm_lib/Body Elements/Revolved Solid  RevolutionCrossSection=[shell_ir 0.5; shell_ir -0.5; shell_or -0.5; shell_or 0.5].*[1 shell_len]  RevolutionCrossSectionUnits=m  RevolutionExtent=Full  RevolutionAngle=180  RevolutionAngleUnits=deg  ExportConvexHullGeometry=off  InertiaType=CalculateFromGeometry  BasedOnType=Density  Density=1  DensityUnits=kg/m^3  Mass=1  MassUnits=kg  CenterOfMass=[0 0 0]  CenterOfMassUnits=m  MomentsOfInertia=[1 1 1]  MomentsOfInertiaUnits=kg*m^2  ProductsOfInertia=[0 0 0]  ProductsOfInertiaUnits=kg*m^2  GraphicType=FromGeometry  MarkerShape=Sphere  MarkerSize=10  GraphicVisPropType=SimpleVisualProperties  GraphicDiffuseColor=shell_clr  GraphicOpacity=shell_opc  GraphicSpecularColor=[0.5 0.5 0.5 1.0]  GraphicAmbientColor=[0.15 0.15 0.15 1.0]  GraphicEmissiveColor=[0.0 0.0 0.0 1.0]  GraphicShininess=75  DoExposeReferenceFrame=on  SerializedFrames=<Frames/>
  Rod : sm_lib/Body Elements/Cylindrical Solid  CylinderRadius=shell_ir/2  CylinderRadiusUnits=m  CylinderLength=shell_len  CylinderLengthUnits=m  ExportEntireGeometry=off  InertiaType=CalculateFromGeometry  BasedOnType=Density  Density=1  DensityUnits=kg/m^3  Mass=1  MassUnits=kg  CenterOfMass=[0 0 0]  CenterOfMassUnits=m  MomentsOfInertia=[1 1 1]  MomentsOfInertiaUnits=kg*m^2  ProductsOfInertia=[0 0 0]  ProductsOfInertiaUnits=kg*m^2  GraphicType=FromGeometry  MarkerShape=Sphere  MarkerSize=10  GraphicVisPropType=SimpleVisualProperties  GraphicDiffuseColor=shell_clr  GraphicOpacity=shell_opc  GraphicSpecularColor=[0.5 0.5 0.5 1.0]  GraphicAmbientColor=[0.15 0.15 0.15 1.0]  GraphicEmissiveColor=[0.0 0.0 0.0 1.0]  GraphicShininess=75  DoExposeReferenceFrame=on  SerializedFrames=<Frames/>
  Transform Align Y Up In : sm_lib/Frames and Transforms/Rigid Transform  RotationMethod=StandardAxis  FollAlignAxisA=+X  BaseAlignAxisA=+Y  FollAlignAxisB=+Y  BaseAlignAxisB=+Z  RotationStandardAxis=+X  RotationAngle=90  RotationAngleUnits=deg  RotationArbitraryAxis=[0 0 1]  RotationSequenceAxes=FollowerAxes  RotationSequence=XYX  RotationSequenceAngles=[0 0 0]  RotationSequenceAnglesUnits=deg  RotationMatrix=[1 0 0; 0 1 0; 0 0 1]  Quaternion=[1 0 0 0]  TranslationMethod=None  TranslationCartesianOffset=[0 0 0]  TranslationCartesianOffsetUnits=m  TranslationStandardAxis=+Z  TranslationStandardOffset=0  TranslationStandardOffsetUnits=m  TranslationROffset=0  TranslationROffsetUnits=m  TranslationThetaOffset=0  TranslationThetaOffsetUnits=deg  TranslationZOffset=0  TranslationZOffsetUnits=m
  Transform Align Y Up Out : sm_lib/Frames and Transforms/Rigid Transform  RotationMethod=StandardAxis  FollAlignAxisA=+X  BaseAlignAxisA=+Y  FollAlignAxisB=+Y  BaseAlignAxisB=+Z  RotationStandardAxis=+X  RotationAngle=90  RotationAngleUnits=deg  RotationArbitraryAxis=[0 0 1]  RotationSequenceAxes=FollowerAxes  RotationSequence=XYX  RotationSequenceAngles=[0 0 0]  RotationSequenceAnglesUnits=deg  RotationMatrix=[1 0 0; 0 1 0; 0 0 1]  Quaternion=[1 0 0 0]  TranslationMethod=None  TranslationCartesianOffset=[0 0 0]  TranslationCartesianOffsetUnits=m  TranslationStandardAxis=+Z  TranslationStandardOffset=0  TranslationStandardOffsetUnits=m  TranslationROffset=0  TranslationROffsetUnits=m  TranslationThetaOffset=0  TranslationThetaOffsetUnits=deg  TranslationZOffset=0  TranslationZOffsetUnits=m
  Triangle : sm_lib/Body Elements/Extruded Solid  ExtrusionType=General  PolygonNumSides=3  PolygonOuterRadius=1  PolygonOuterRadiusUnits=m  ExportEntireGeometry=off  ExtrusionCrossSection=[cosd(-70) sind(-70);1 0;cosd(70) sind(70)]*shell_or  ExtrusionCrossSectionUnits=m  ExportConvexHullGeometry=off  ExtrusionLength=shell_len+0.001  ExtrusionLengthUnits=m  InertiaType=CalculateFromGeometry  BasedOnType=Density  Density=1  DensityUnits=kg/m^3  Mass=1  MassUnits=kg  CenterOfMass=[0 0 0]  CenterOfMassUnits=m  MomentsOfInertia=[1 1 1]  MomentsOfInertiaUnits=kg*m^2  ProductsOfInertia=[0 0 0]  ProductsOfInertiaUnits=kg*m^2  GraphicType=FromGeometry  MarkerShape=Sphere  MarkerSize=10  GraphicVisPropType=SimpleVisualProperties  GraphicDiffuseColor=[0.6 1.0 0.0]  GraphicOpacity=1.0  GraphicSpecularColor=[0.5 0.5 0.5 1.0]  GraphicAmbientColor=[0.15 0.15 0.15 1.0]  GraphicEmissiveColor=[0.0 0.0 0.0 1.0]  GraphicShininess=75  DoExposeReferenceFrame=on  SerializedFrames=<Frames/>
  Universal Joint : sm_lib/Joints/Universal Joint  JointMode=Normal  CompositeWrenchDir=FollowerOnBase  CompositeWrenchFrame=BaseFrame  SenseConstraintForce=off  SenseConstraintTorque=off  SenseTotalForce=off  SenseTotalTorque=off  RxPositionTargetSpecify=off  RxPositionTargetPriority=High  RxPositionTargetValue=0  RxPositionTargetValueUnits=deg  RxVelocityTargetSpecify=off  RxVelocityTargetPriority=High  RxVelocityTargetValue=0  RxVelocityTargetValueUnits=deg/s  RxEquilibriumPosition=0  RxEquilibriumPositionUnits=deg  RxSpringStiffness=0  RxSpringStiffnessUnits=N*m/deg  RxDampingCoefficient=0  RxDampingCoefficientUnits=N*m/(deg/s)  RxLowerLimitSpecify=off  RxLowerLimitBound=-90  RxLowerLimitBoundUnits=deg  RxLowerLimitStiffness=1e4  RxLowerLimitStiffnessUnits=N*m/deg  RxLowerLimitDamping=10  RxLowerLimitDampingUnits=N*m/(deg/s)  RxLowerLimitTransitionRegionWidth=0.1  RxLowerLimitTransitionRegionWidthUnits=deg  RxUpperLimitSpecify=off  RxUpperLimitBound=90  RxUpperLimitBoundUnits=deg  RxUpperLimitStiffness=1e4  RxUpperLimitStiffnessUnits=N*m/deg  RxUpperLimitDamping=10  RxUpperLimitDampingUnits=N*m/(deg/s)  RxUpperLimitTransitionRegionWidth=0.1  RxUpperLimitTransitionRegionWidthUnits=deg  RxTorqueActuationMode=NoTorque  RxMotionActuationMode=ComputedMotion  RxSensePosition=off  RxSenseVelocity=off  RxSenseAcceleration=off  RxSenseTorqueForce=off  RxSenseLowerLimitTorqueForce=off  RxSenseUpperLimitTorqueForce=off  RyPositionTargetSpecify=off  RyPositionTargetPriority=High  RyPositionTargetValue=0  RyPositionTargetValueUnits=deg  RyVelocityTargetSpecify=off  RyVelocityTargetPriority=High  RyVelocityTargetValue=0  RyVelocityTargetValueUnits=deg/s  RyEquilibriumPosition=0  RyEquilibriumPositionUnits=deg  RySpringStiffness=0  RySpringStiffnessUnits=N*m/deg  RyDampingCoefficient=0  RyDampingCoefficientUnits=N*m/(deg/s)  RyLowerLimitSpecify=off  RyLowerLimitBound=-90  RyLowerLimitBoundUnits=deg  RyLowerLimitStiffness=1e4  RyLowerLimitStiffnessUnits=N*m/deg  RyLowerLimitDamping=10  RyLowerLimitDampingUnits=N*m/(deg/s)  RyLowerLimitTransitionRegionWidth=0.1  RyLowerLimitTransitionRegionWidthUnits=deg  RyUpperLimitSpecify=off  RyUpperLimitBound=90  RyUpperLimitBoundUnits=deg  RyUpperLimitStiffness=1e4  RyUpperLimitStiffnessUnits=N*m/deg  RyUpperLimitDamping=10  RyUpperLimitDampingUnits=N*m/(deg/s)  RyUpperLimitTransitionRegionWidth=0.1  RyUpperLimitTransitionRegionWidthUnits=deg  RyTorqueActuationMode=NoTorque  RyMotionActuationMode=ComputedMotion  RySensePosition=off  RySenseVelocity=off  RySenseAcceleration=off  RySenseTorqueForce=off  RySenseLowerLimitTorqueForce=off  RySenseUpperLimitTorqueForce=off
  B : PMIOPort  Side=Left
  F : PMIOPort  Port=2  Side=Right
  m : Outport
  wires:
  Force Law/1 -> m/1
  connections:
  Bushing Joint/LConn3 -- Force Law/LConn2
  Outer Shell/RConn1 -- Bushing Joint/RConn1 -- Transform Align Y Up Out/LConn1 -- Triangle/RConn1
  Bushing Joint/RConn3 -- Force Law/RConn5
  Bushing Joint/LConn2 -- Force Law/LConn3
  Bushing Joint/LConn4 -- Force Law/LConn1
  Bushing Joint/RConn7 -- Force Law/RConn1
  Bushing Joint/RConn5 -- Force Law/RConn3
  Bushing Joint/RConn6 -- Force Law/RConn2
  Bushing Joint/RConn4 -- Force Law/RConn4
  Bushing Joint/RConn2 -- Force Law/RConn6
  Rod/RConn1 -- Bushing Joint/LConn1 -- B/RConn1
  Transform Align Y Up Out/RConn1 -- Universal Joint/LConn1
  Universal Joint/RConn1 -- Transform Align Y Up In/RConn1
  F/RConn1 -- Transform Align Y Up In/LConn1
